simulink model "Rl_toy"  (R2025b)
settings: Solver=VariableStepAuto  StartTime=0.0  StopTime=5000  RelTol=1e-3
values from neighbouring files (symbols this model uses):
  Rc_alu = 10    [modele_valeur.m]
  Rc_fan = 1.2/2    (= 0.6)    [modele_valeur.m]
  Rc_fan1 = 1.2/2    (= 0.6)    [modele_valeur.m]
  Rc_pet = 20/2    (= 10)    [modele_valeur.m]
  Rc_pet1 = 20/2    (= 10)    [modele_valeur.m]
  Rth_alu = 0.1/2    (= 0.05)    [modele_valeur.m]
  Rth_alu2 = 0.1/2    (= 0.05)    [modele_valeur.m]
  Rth_fan = 2.5/2    (= 1.25)    [modele_valeur.m]
  Rth_fan2 = 2.5/2    (= 1.25)    [modele_valeur.m]
  Rth_pet = 5/2    (= 2.5)    [modele_valeur.m]
  Rth_pet2 = 5/2    (= 2.5)    [modele_valeur.m]
  Rth_sen = 24    [modele_valeur.m]
  Rv_max = 50    [thermal_rl_env.m]
  Rv_min = 0.02    [thermal_rl_env.m]
  Ts = 1    [model_file_elec.m]    (also in modele_valeur.m; thermal_rl_env.m = 0.5)
libraries: fl_lib x33, nesl_utility x6, rllib x1
settings Model: Creator=aymoun  LastModifiedBy=nael

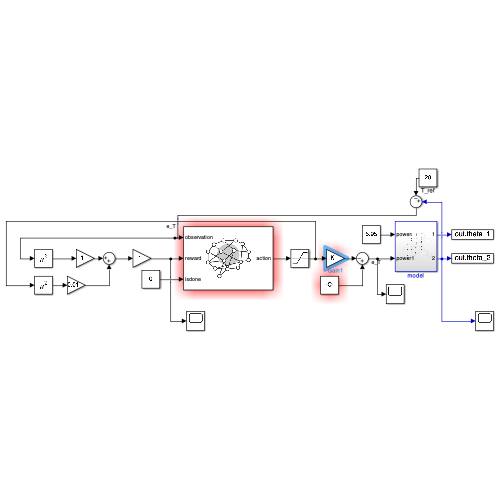
[thumbnail: Simulink's stored preview of the top-level diagram]
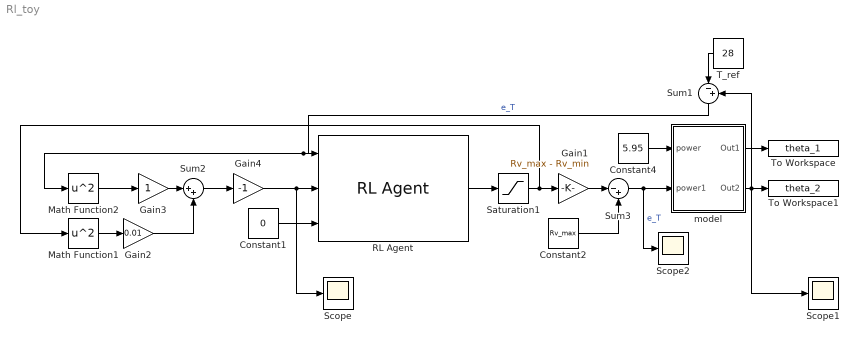
== system Rl_toy ==
  Constant1 : Constant  Value=0
  Constant2 : Constant  Value=Rv_max  SampleTime=Ts
  Constant4 : Constant  Value=5.95  SampleTime=Ts
  Gain1 : Gain  Gain=Rv_max - Rv_min
  Gain2 : Gain  Gain=0.01
  Gain3 : Gain
  Gain4 : Gain  Gain=-1
  Math Function1 : Math  Operator=square
  Math Function2 : Math  Operator=square
  RL Agent : rllib/RL Agent  Agent=agent  ExternalActionAsInput=off  ProvideLastAction=off  ProvideCumRwd=off  TreatAsDirectFeedthrough=on  UseStrictObservationDataTypes=off
  Saturation1 : Saturate  UpperLimit=1  LowerLimit=0
  Scope : Scope
      settings: ActiveDisplayYMinimum=-38.93561  ActiveDisplayYMaximum=4.32618
  Scope1 : Scope
      settings: ActiveDisplayYMinimum=13.497710861966819  ActiveDisplayYMaximum=34.11774163042876  DataLoggingVariableName=ScopeData2
  Scope2 : Scope
      settings: ActiveDisplayYMinimum=-1  ActiveDisplayYMaximum=1  DataLoggingVariableName=ScopeData2
  Sum1 : Sum  Inputs=|-+
  Sum2 : Sum  Inputs=|++
  Sum3 : Sum  Inputs=|-+
  T_ref : Constant  Value=28  SampleTime=Ts
  To Workspace : ToWorkspace  VariableName=theta_1  SampleTime=-1
  To Workspace1 : ToWorkspace  VariableName=theta_2  SampleTime=Ts
  model : Subsystem
  wires:
  model/1(Out1) -> To Workspace/1
  model/2(Out2) -> Scope1/1, Sum1/2, To Workspace1/1
  T_ref/1 -> Sum1/1
  Constant1/1 -> RL Agent/3
  Sum1/1 -> Math Function2/1, RL Agent/1  "e_T"
  Math Function1/1 -> Gain2/1
  Math Function2/1 -> Gain3/1
  Gain4/1 -> RL Agent/2, Scope/1
  Sum2/1 -> Gain4/1
  Constant2/1 -> Sum3/2
  Gain1/1 -> Sum3/1
  Sum3/1 -> model/2(power1), Scope2/1  "e_T"
  Constant4/1 -> model/1(power)
  RL Agent/1 -> Saturation1/1
  Gain2/1 -> Sum2/2
  Gain3/1 -> Sum2/1
  Saturation1/1 -> Gain1/1, Math Function1/1

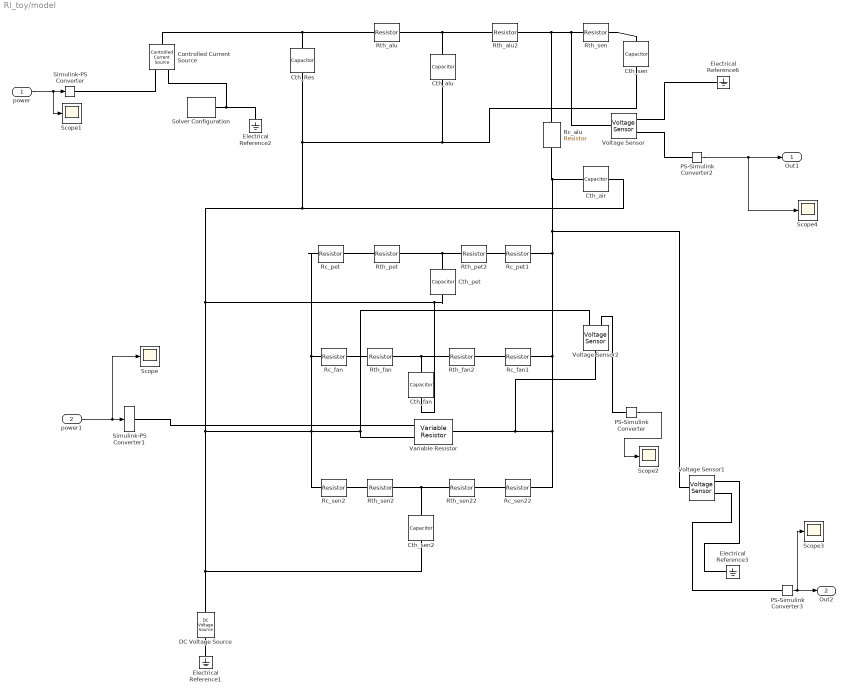
== system Rl_toy/model ==
  power : Inport
  power1 : Inport  Port=2
  Controlled Current Source : fl_lib/Electrical/Electrical Sources/Controlled Current Source
  Cth_Res : fl_lib/Electrical/Electrical Elements/Capacitor  c=Cth_Res F  r=0 Ohm  g=0 1/Ohm  i_specify=off  i_priority=None  i=0 A  i_nominal_specify=off  i_nominal_value=1  i_nominal_unit=A  v_specify=off  v_priority=None  v=0 V  v_nominal_specify=off  v_nominal_value=1  v_nominal_unit=V  vc_specify=off  vc_priority=High  vc=0 V  vc_nominal_specify=off  vc_nominal_value=1  vc_nominal_unit=V
  Cth_air : fl_lib/Electrical/Electrical Elements/Capacitor  c=Cth_air F  r=0 Ohm  g=0 1/Ohm  i_specify=off  i_priority=None  i=0 A  i_nominal_specify=off  i_nominal_value=1  i_nominal_unit=A  v_specify=off  v_priority=None  v=0 V  v_nominal_specify=off  v_nominal_value=1  v_nominal_unit=V  vc_specify=off  vc_priority=High  vc=0 V  vc_nominal_specify=off  vc_nominal_value=1  vc_nominal_unit=V
  Cth_alu : fl_lib/Electrical/Electrical Elements/Capacitor  c=Cth_alu F  r=0 Ohm  g=0 1/Ohm  i_specify=off  i_priority=None  i=0 A  i_nominal_specify=off  i_nominal_value=1  i_nominal_unit=A  v_specify=off  v_priority=None  v=0 V  v_nominal_specify=off  v_nominal_value=1  v_nominal_unit=V  vc_specify=off  vc_priority=High  vc=0 V  vc_nominal_specify=off  vc_nominal_value=1  vc_nominal_unit=V
  Cth_fan : fl_lib/Electrical/Electrical Elements/Capacitor  c=Cth_fan F  r=0 Ohm  g=0 1/Ohm  i_specify=off  i_priority=None  i=0 A  i_nominal_specify=off  i_nominal_value=1  i_nominal_unit=A  v_specify=off  v_priority=None  v=0 V  v_nominal_specify=off  v_nominal_value=1  v_nominal_unit=V  vc_specify=off  vc_priority=High  vc=0 V  vc_nominal_specify=off  vc_nominal_value=1  vc_nominal_unit=V
  Cth_pet : fl_lib/Electrical/Electrical Elements/Capacitor  c=Cth_pet F  r=0 Ohm  g=0 1/Ohm  i_specify=off  i_priority=None  i=0 A  i_nominal_specify=off  i_nominal_value=1  i_nominal_unit=A  v_specify=off  v_priority=None  v=0 V  v_nominal_specify=off  v_nominal_value=1  v_nominal_unit=V  vc_specify=off  vc_priority=High  vc=0 V  vc_nominal_specify=off  vc_nominal_value=1  vc_nominal_unit=V
  Cth_sen : fl_lib/Electrical/Electrical Elements/Capacitor  c=Cth_sen F  r=0 Ohm  g=0 1/Ohm  i_specify=off  i_priority=None  i=0 A  i_nominal_specify=off  i_nominal_value=1  i_nominal_unit=A  v_specify=off  v_priority=None  v=0 V  v_nominal_specify=off  v_nominal_value=1  v_nominal_unit=V  vc_specify=off  vc_priority=High  vc=0 V  vc_nominal_specify=off  vc_nominal_value=1  vc_nominal_unit=V
  Cth_sen2 : fl_lib/Electrical/Electrical Elements/Capacitor  c=Cth_pet F  r=0 Ohm  g=0 1/Ohm  i_specify=off  i_priority=None  i=0 A  i_nominal_specify=off  i_nominal_value=1  i_nominal_unit=A  v_specify=off  v_priority=None  v=0 V  v_nominal_specify=off  v_nominal_value=1  v_nominal_unit=V  vc_specify=off  vc_priority=High  vc=0 V  vc_nominal_specify=off  vc_nominal_value=1  vc_nominal_unit=V
  DC Voltage Source : fl_lib/Electrical/Electrical Sources/DC Voltage Source  v0=22 V
  Electrical Reference{1..3,6} (4 alike) : fl_lib/Electrical/Electrical Elements/Electrical Reference
  PS-Simulink Converter : nesl_utility/PS-Simulink Converter  PhysicalDomain=network_engine_domain  SubClassName=ps_output  LeftPortType=input  RightPortType=output  PseudoPeriodic=off  Frequencies=[]  VectorFormat=inherit  Unit=inherit  AffineConversion=off
  PS-Simulink Converter2 : nesl_utility/PS-Simulink Converter  PhysicalDomain=network_engine_domain  SubClassName=ps_output  LeftPortType=input  RightPortType=output  PseudoPeriodic=off  Frequencies=[]  VectorFormat=inherit  Unit=inherit  AffineConversion=off
  PS-Simulink Converter3 : nesl_utility/PS-Simulink Converter  PhysicalDomain=network_engine_domain  SubClassName=ps_output  LeftPortType=input  RightPortType=output  PseudoPeriodic=off  Frequencies=[]  VectorFormat=inherit  Unit=inherit  AffineConversion=off
  Rc_alu : fl_lib/Electrical/Electrical Elements/Resistor  R=Rc_alu Ohm  i_specify=off  i_priority=None  i=0 A  i_nominal_specify=off  i_nominal_value=1  i_nominal_unit=A  v_specify=off  v_priority=None  v=0 V  v_nominal_specify=off  v_nominal_value=1  v_nominal_unit=V
  Rc_fan : fl_lib/Electrical/Electrical Elements/Resistor  R=Rc_fan Ohm  i_specify=off  i_priority=None  i=0 A  i_nominal_specify=off  i_nominal_value=1  i_nominal_unit=A  v_specify=off  v_priority=None  v=0 V  v_nominal_specify=off  v_nominal_value=1  v_nominal_unit=V
  Rc_fan1 : fl_lib/Electrical/Electrical Elements/Resistor  R=Rc_fan1 Ohm  i_specify=off  i_priority=None  i=0 A  i_nominal_specify=off  i_nominal_value=1  i_nominal_unit=A  v_specify=off  v_priority=None  v=0 V  v_nominal_specify=off  v_nominal_value=1  v_nominal_unit=V
  Rc_pet : fl_lib/Electrical/Electrical Elements/Resistor  R=Rc_pet Ohm  i_specify=off  i_priority=None  i=0 A  i_nominal_specify=off  i_nominal_value=1  i_nominal_unit=A  v_specify=off  v_priority=None  v=0 V  v_nominal_specify=off  v_nominal_value=1  v_nominal_unit=V
  Rc_pet1 : fl_lib/Electrical/Electrical Elements/Resistor  R=Rc_pet1 Ohm  i_specify=off  i_priority=None  i=0 A  i_nominal_specify=off  i_nominal_value=1  i_nominal_unit=A  v_specify=off  v_priority=None  v=0 V  v_nominal_specify=off  v_nominal_value=1  v_nominal_unit=V
  Rc_sen2 : fl_lib/Electrical/Electrical Elements/Resistor  R=Rc_fan Ohm  i_specify=off  i_priority=None  i=0 A  i_nominal_specify=off  i_nominal_value=1  i_nominal_unit=A  v_specify=off  v_priority=None  v=0 V  v_nominal_specify=off  v_nominal_value=1  v_nominal_unit=V
  Rc_sen22 : fl_lib/Electrical/Electrical Elements/Resistor  R=Rth_fan Ohm  i_specify=off  i_priority=None  i=0 A  i_nominal_specify=off  i_nominal_value=1  i_nominal_unit=A  v_specify=off  v_priority=None  v=0 V  v_nominal_specify=off  v_nominal_value=1  v_nominal_unit=V
  Rth_alu : fl_lib/Electrical/Electrical Elements/Resistor  R=Rth_alu Ohm  i_specify=off  i_priority=None  i=0 A  i_nominal_specify=off  i_nominal_value=1  i_nominal_unit=A  v_specify=off  v_priority=None  v=0 V  v_nominal_specify=off  v_nominal_value=1  v_nominal_unit=V
  Rth_alu2 : fl_lib/Electrical/Electrical Elements/Resistor  R=Rth_alu2 Ohm  i_specify=off  i_priority=None  i=0 A  i_nominal_specify=off  i_nominal_value=1  i_nominal_unit=A  v_specify=off  v_priority=None  v=0 V  v_nominal_specify=off  v_nominal_value=1  v_nominal_unit=V
  Rth_fan : fl_lib/Electrical/Electrical Elements/Resistor  R=Rth_fan Ohm  i_specify=off  i_priority=None  i=0 A  i_nominal_specify=off  i_nominal_value=1  i_nominal_unit=A  v_specify=off  v_priority=None  v=0 V  v_nominal_specify=off  v_nominal_value=1  v_nominal_unit=V
  Rth_fan2 : fl_lib/Electrical/Electrical Elements/Resistor  R=Rth_fan2 Ohm  i_specify=off  i_priority=None  i=0 A  i_nominal_specify=off  i_nominal_value=1  i_nominal_unit=A  v_specify=off  v_priority=None  v=0 V  v_nominal_specify=off  v_nominal_value=1  v_nominal_unit=V
  Rth_pet : fl_lib/Electrical/Electrical Elements/Resistor  R=Rth_pet Ohm  i_specify=off  i_priority=None  i=0 A  i_nominal_specify=off  i_nominal_value=1  i_nominal_unit=A  v_specify=off  v_priority=None  v=0 V  v_nominal_specify=off  v_nominal_value=1  v_nominal_unit=V
  Rth_pet2 : fl_lib/Electrical/Electrical Elements/Resistor  R=Rth_pet2 Ohm  i_specify=off  i_priority=None  i=0 A  i_nominal_specify=off  i_nominal_value=1  i_nominal_unit=A  v_specify=off  v_priority=None  v=0 V  v_nominal_specify=off  v_nominal_value=1  v_nominal_unit=V
  Rth_sen : fl_lib/Electrical/Electrical Elements/Resistor  R=Rth_sen Ohm  i_specify=off  i_priority=None  i=0 A  i_nominal_specify=off  i_nominal_value=1  i_nominal_unit=A  v_specify=off  v_priority=None  v=0 V  v_nominal_specify=off  v_nominal_value=1  v_nominal_unit=V
  Rth_sen2 : fl_lib/Electrical/Electrical Elements/Resistor  R=Rth_fan Ohm  i_specify=off  i_priority=None  i=0 A  i_nominal_specify=off  i_nominal_value=1  i_nominal_unit=A  v_specify=off  v_priority=None  v=0 V  v_nominal_specify=off  v_nominal_value=1  v_nominal_unit=V
  Rth_sen22 : fl_lib/Electrical/Electrical Elements/Resistor  R=Rc_fan Ohm  i_specify=off  i_priority=None  i=0 A  i_nominal_specify=off  i_nominal_value=1  i_nominal_unit=A  v_specify=off  v_priority=None  v=0 V  v_nominal_specify=off  v_nominal_value=1  v_nominal_unit=V
  Scope{,1..4} (5 alike) : Scope
      Scope settings: ActiveDisplayYMinimum=0.01  ActiveDisplayYMaximum=0.03
      Scope1 settings: ActiveDisplayYMinimum=21.999999988  ActiveDisplayYMaximum=22.000000012
      Scope2 settings: ActiveDisplayYMinimum=-7E-17  ActiveDisplayYMaximum=5E-17
      Scope3 settings: ActiveDisplayYMinimum=12  ActiveDisplayYMaximum=32  DataLoggingVariableName=ScopeData2
      Scope4 settings: ActiveDisplayYMinimum=14.43347  ActiveDisplayYMaximum=90.0988  DataLoggingVariableName=ScopeData4
  Simulink-PS Converter : nesl_utility/Simulink-PS Converter  PhysicalDomain=network_engine_domain  SubClassName=ps_input  LeftPortType=input  RightPortType=output  PseudoPeriodic=off  Frequencies=[]  NoiseDistribution=none  NoiseParameters=[]  Unit=1  AffineConversion=off  FilteringAndDerivatives=provide  SimscapeFilterOrder=1  InputFilterTimeConstant=0.001  UdotUserProvided=0
  Simulink-PS Converter1 : nesl_utility/Simulink-PS Converter  PhysicalDomain=network_engine_domain  SubClassName=ps_input  LeftPortType=input  RightPortType=output  PseudoPeriodic=off  Frequencies=[]  NoiseDistribution=none  NoiseParameters=[]  Unit=V/A  AffineConversion=off  FilteringAndDerivatives=filter  SimscapeFilterOrder=1  InputFilterTimeConstant=Ts  UdotUserProvided=0
  Solver Configuration : nesl_utility/Solver Configuration  PhysicalDomain=network_engine_domain  SubClassName=solver  LeftPortType=input  RightPortType=generic  Tones=[]  Harmonics=[]  SimulateNoise=off  Profile=off  UseLocalSampling=off  EnableSwitchedLinearOptims=on  FrequencyDomain=off  UseCCode=off  RelTol=0.001  AbsTol=0.001  MinStep=1e-09  ToWorkspace=off  RevertToSquareIcSolve=off  NumHomotopyIterations=100  PhasorMode=off  PhasorModeNumHarmonics=1  ConsistencySolver=NEWTON_XTOL_AFTER_FTOL  IndexReductionMethod=DerivativeReplacement  DoDC=off  ResidualTolerance=1e-09  ConsistencyTolSource=GLOBAL  ConsistencyAbsTol=0.001  ConsistencyRelTol=0.001  ConsistencyTolFactor=0.001  UseLocalSolver=off  LocalSolverChoice=NE_BACKWARD_EULER_ADVANCER  ResolveIndetEquations=on  FunctionEvalNumThread=1  LocalSolverSampleTime=0.001  DoFixedCost=off  MaxNonlinIter=3  MaxModeIter=2  ComputeImpulses=off  ImpulseIterations=2  LinearAlgebra=auto  LinearAlgebraNumThread=0  EquationFormulation=NE_TIME_EF  DelaysMemoryBudget=1024  AutomaticFiltering=on  FilteringTimeConstant=0.001  PartitionStorageMethod=AS_NEEDED  PartitionMemoryBudget=1024  PartitionMethod=ROBUST  MultibodyUseLocalSolver=off  MultibodyLocalSolverChoice=ODE1  MultibodyLocalSolverSampleTime=0.001
  Variable Resistor : fl_lib/Electrical/Electrical Elements/Variable Resistor  Rmin=0.2 Ohm  thermalEnable=false  thermal_mass=1 J/K  i_specify=off  i_priority=None  i=0 A  i_nominal_specify=off  i_nominal_value=1  i_nominal_unit=A  v_specify=off  v_priority=None  v=0 V  v_nominal_specify=off  v_nominal_value=1  v_nominal_unit=V  T_specify=off  T_priority=None  T=300 K  T_nominal_specify=off  T_nominal_value=1  T_nominal_unit=K
  Voltage Sensor : fl_lib/Electrical/Electrical Sensors/Voltage Sensor
  Voltage Sensor1 : fl_lib/Electrical/Electrical Sensors/Voltage Sensor
  Voltage Sensor2 : fl_lib/Electrical/Electrical Sensors/Voltage Sensor
  Out1 : Outport
  Out2 : Outport  Port=2
  wires:
  PS-Simulink Converter3/1 -> Scope3/1, Out2/1
  PS-Simulink Converter2/1 -> Scope4/1, Out1/1
  power/1 -> Scope1/1, Simulink-PS Converter/1
  PS-Simulink Converter/1 -> Scope2/1
  power1/1 -> Scope/1, Simulink-PS Converter1/1
  connections:
  Cth_Res/RConn1 -- Cth_sen/RConn1 -- Cth_alu/RConn1 -- Cth_air/RConn1 -- Cth_fan/RConn1 -- Cth_pet/RConn1 -- DC Voltage Source/LConn1 -- Cth_sen2/RConn1 -- Rc_sen2/LConn1 -- Rc_pet/LConn1 -- Rc_fan/LConn1 -- Variable Resistor/LConn2 -- Voltage Sensor2/RConn2
  Voltage Sensor/LConn1 -- Rth_alu2/RConn1 -- Rc_alu/LConn1 -- Rth_sen/LConn1
  Rth_pet/RConn1 -- Cth_pet/LConn1 -- Rth_pet2/LConn1
  Rth_fan2/LConn1 -- Cth_fan/LConn1 -- Rth_fan/RConn1
  Cth_alu/LConn1 -- Rth_alu2/LConn1 -- Rth_alu/RConn1
  Cth_Res/LConn1 -- Controlled Current Source/LConn1 -- Rth_alu/LConn1
  Solver Configuration/RConn1 -- Controlled Current Source/RConn2 -- Electrical Reference2/LConn1
  Rth_sen22/LConn1 -- Rth_sen2/RConn1 -- Cth_sen2/LConn1
  Electrical Reference3/LConn1 -- Voltage Sensor1/RConn2
  DC Voltage Source/RConn1 -- Electrical Reference1/LConn1
  Rth_sen/RConn1 -- Cth_sen/LConn1
  Rth_pet/LConn1 -- Rc_pet/RConn1
  Voltage Sensor1/RConn1 -- PS-Simulink Converter3/LConn1
  Rth_fan/LConn1 -- Rc_fan/RConn1
  Rth_sen2/LConn1 -- Rc_sen2/RConn1
  Controlled Current Source/RConn1 -- Simulink-PS Converter/RConn1
  Electrical Reference6/LConn1 -- Voltage Sensor/RConn2
  Rc_sen22/LConn1 -- Rth_sen22/RConn1
  Rc_fan1/LConn1 -- Rth_fan2/RConn1
  Voltage Sensor/RConn1 -- PS-Simulink Converter2/LConn1
  Rc_pet1/LConn1 -- Rth_pet2/RConn1
  Voltage Sensor1/LConn1 -- Cth_air/LConn1 -- Rc_alu/RConn1 -- Rc_pet1/RConn1 -- Rc_fan1/RConn1 -- Rc_sen22/RConn1 -- Voltage Sensor2/LConn1 -- Variable Resistor/RConn1
  Voltage Sensor2/RConn1 -- PS-Simulink Converter/LConn1
  Variable Resistor/LConn1 -- Simulink-PS Converter1/RConn1
